simulink model "pcssp_controller_and_ps_psc"  (R2025b)
settings: Solver=VariableStepAuto  StartTime=t_start  StopTime=t_max  RelTol=1e-3
values from neighbouring files (symbols this model uses):
  AllocatorMode = 1    [muscle_controller_NICE_IMAS_iter_init.m]    (also in muscle_controller_NICE_IMAS_iter_init_psc.m)
  enable_KCURR = double(instance.get_setting('KCURR', pyargs('default', 1)))    [muscle_controller_NICE_IMAS_iter_init.m]    (also in muscle_controller_NICE_IMAS_iter_init_psc.m)
  enable_RZIp = double(instance.get_setting('RZIp', pyargs('default', 0)))    [muscle_controller_NICE_IMAS_iter_init.m]    (also in muscle_controller_NICE_IMAS_iter_init_psc.m)
  enable_VS = double(instance.get_setting('VS', pyargs('default', 1)))    [muscle_controller_NICE_IMAS_iter_init.m]    (also in muscle_controller_NICE_IMAS_iter_init_psc.m)
  in_out_dt = double(instance.get_setting('in_out_msg_dt', pyargs('default', 0.001)))    [muscle_controller_NICE_IMAS_iter_init.m]    (also in muscle_controller_NICE_IMAS_iter_init_psc.m)
  IpControlMode = 0    [muscle_controller_NICE_IMAS_iter_init.m]    (also in muscle_controller_NICE_IMAS_iter_init_psc.m)
  IpControlMode_KCURR = double(instance.get_setting('control_Ip', pyargs('default', 1)))    [muscle_controller_NICE_IMAS_iter_init.m]    (also in muscle_controller_NICE_IMAS_iter_init_psc.m)
  IpControlMode_RZIp = 0    [muscle_controller_NICE_IMAS_iter_init.m]    (also in muscle_controller_NICE_IMAS_iter_init_psc.m)
  SchedulingVar_GapContr = 0    [muscle_controller_NICE_IMAS_iter_init.m]    (also in muscle_controller_NICE_IMAS_iter_init_psc.m)
  schedulingVar_KCURR = 0    [muscle_controller_NICE_IMAS_iter_init.m]    (also in muscle_controller_NICE_IMAS_iter_init_psc.m)
  SCIpScaling = 0    [muscle_controller_NICE_IMAS_iter_init.m]    (also in muscle_controller_NICE_IMAS_iter_init_psc.m)
  ShapeIpControlMode = double(instance.get_setting('Shape_control', pyargs('default', 0)))    [muscle_controller_NICE_IMAS_iter_init.m]    (also in muscle_controller_NICE_IMAS_iter_init_psc.m)
  usePSModel = double(instance.get_setting('PSModel', pyargs('default', 1)))    [muscle_controller_NICE_IMAS_iter_init.m]    (also in muscle_controller_NICE_IMAS_iter_init_psc.m)
  VSControlMode = double(instance.get_setting('VS_control_mode', pyargs('default', 3)))    [muscle_controller_NICE_IMAS_iter_init.m]    (also in muscle_controller_NICE_IMAS_iter_init_psc.m)
  VSIpScaling = 1    [muscle_controller_NICE_IMAS_iter_init.m]    (also in muscle_controller_NICE_IMAS_iter_init_psc.m)
Description:
  | The KCURR_PFPO1 module implements a CS/PF current controller, including control of IpThis version performs internal gain scheduling based on an externally fed scheduling variable. Note: the coils are sorted as CS3U CS2U CS1 CS2L CS3L P1 P2 P3 P4 P5 P6
settings Model: DataDictionary=pcssp_controller_and_ps_psc.sldd  VariantFading=off  Creator=ravenst1  LastModifiedBy=schneim
settings SolverCC: AutoInsertRateTranBlk=on
settings DebuggingCC: UnderspecifiedInitializationDetection=Classic  MergeDetectMultiDrivingBlocksExec=none
settings ModelReferenceCC: PropagateSignalLabelsOutOfModel=off

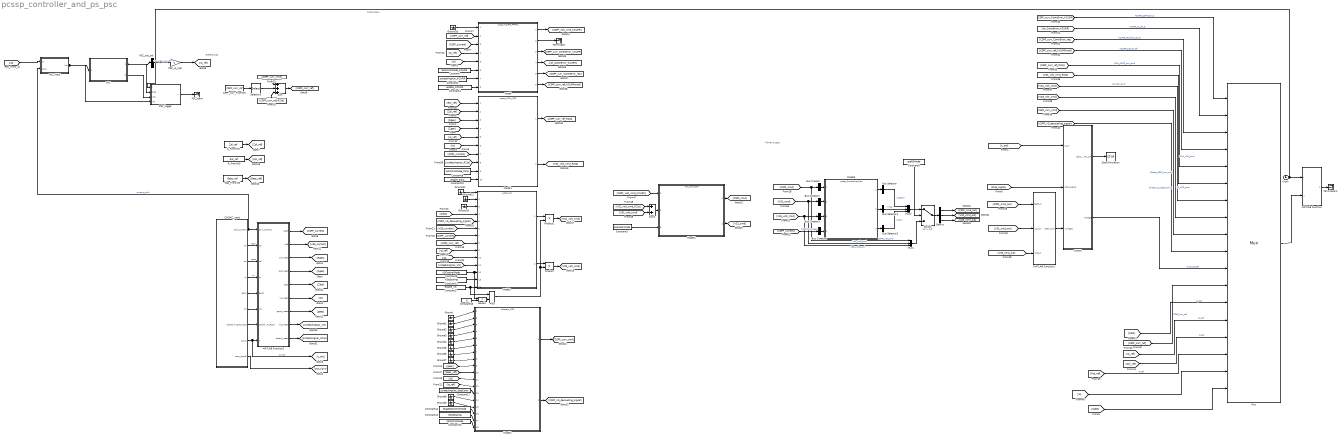
== system pcssp_controller_and_ps_psc ==
  note: Power supply
  note: Controllers
  note: References
  AND : Logic  IconShape=distinctive  AllPortsSameDT=off  OutDataTypeStr=boolean
  Bus Creator : BusCreator  Inputs=1  OutDataTypeStr=Bus:pcssp_PS_CSPF_volt_cmd
  Bus Creator2 : BusCreator  Inputs=1  OutDataTypeStr=Bus: pcssp_PS_VS1_volt_cmd
  Bus Creator3 : BusCreator  Inputs=1  OutDataTypeStr=Bus: pcssp_PS_VS3_volt_cmd
  Bus Creator4 : BusCreator  Inputs=1  OutDataTypeStr=Bus: pcssp_PS_CSPF_curr_meas
  Bus Selector : BusSelector  OutputSignals=VCSPF
  Bus Selector1 : BusSelector  OutputSignals=VS1
  Bus Selector2 : BusSelector  OutputSignals=VS3
  CODAC_input : MATLAB Function  TreatAsAtomicUnit=on  SystemSampleTime=in_out_dt
  CSPF_curr_FromWS : FromWorkspace  VariableName=CSPF_curr_ref
  Clock : Clock
  Constant : Constant  Value=IpControlMode_KCURR  OutDataTypeStr=boolean
  Constant1 : Constant  Value=schedulingVar_KCURR
  Constant10 : Constant  Value=enable_RZIp  OutDataTypeStr=boolean
  Constant11 : Constant  Value=VSIpScaling
  Constant12 : Constant  Value=SCIpScaling
  Constant13 : Constant  Value=IpControlMode
  Constant14 : Constant  Value=ShapeIpControlMode
  Constant15 : Constant  Value=0
  Constant17 : Constant  Value=SchedulingVar_GapContr
  Constant2 : Constant  Value=enable_VS  OutDataTypeStr=boolean
  Constant3 : Constant  Value=AllocatorMode
  Constant4 : Constant  Value=enable_KCURR
  Constant5 : Constant  Value=usePSModel
  Constant6 : Constant  Value=VSControlMode
  Constant8 : Constant  Value=IpControlMode_RZIp  OutDataTypeStr=boolean
  Demux : Demux  Outputs=[11 1 1]
  Equal4 : RelationalOperator  Operator=>  OutDataTypeStr=boolean  RndMeth=Simplest  InputSameDT=off
  Gap_FromWS : FromWorkspace  VariableName=Gaps_ref
  Ground{,1..13} (14 alike) : Ground
  MATLAB Function : MATLAB Function  TreatAsAtomicUnit=on  SystemSampleTime=in_out_dt
  MATLAB Function1 : MATLAB Function  TreatAsAtomicUnit=on  SystemSampleTime=in_out_dt
  MATLAB Function2 : MATLAB Function  TreatAsAtomicUnit=on  SystemSampleTime=in_out_dt
  Model : ModelReference  ModelNameDialog=pcssp_KCURR_PFPO1.slx  SimulationMode=Normal  ModelReferenceVersion=6.1
  Model1 : ModelReference  ModelNameDialog=pcssp_RZIp_CCS.slx  SimulationMode=Normal  ModelReferenceVersion=10.5
  Model2 : ModelReference  ModelNameDialog=shapeIp_CCS.slx  SimulationMode=Normal  ModelReferenceVersion=1.1
  Model3 : ModelReference  ModelNameDialog=pcssp_VS.slx  SimulationMode=Normal  ModelReferenceVersion=7.2
  Model4 : ModelReference  ModelNameDialog=VS1_allocator.slx  SimulationMode=Normal  ModelReferenceVersion=1.4
  Model5 : ModelReference  ModelNameDialog=pcssp_PowerSupplies.slx  ParameterArgumentNames=PS_tp  UsingDefaultArgumentValue=0  SimulationMode=Normal  ModelReferenceVersion=1.39
  Mux : Mux  Inputs=18
      settings: DisplayOption=signals
  Mux1 : Mux  Inputs=3
  Mux2 : Mux  Inputs=3
  Output : MATLAB Function  TreatAsAtomicUnit=on  SystemSampleTime=in_out_dt
  PSC : Subsystem  ReferencedSubsystem=PSC  ConfFolderPath=/Users/igo/Data_Igor_Local/GitFolder/pcs  PSCInterConfFileName=[]  GlobMonFileName=[]  DecisionFileName=[]  RefGenFileName=[]  useInBus=Bus signal  useInPorts=Ports  useOutBus=Bus signal  useOutPorts=Ports  SaveStatus=off
  PSC_Ip_sign : Gain  Gain=-1
  PSC_input : MATLAB Function  TreatAsAtomicUnit=on
  PSC_logger : MATLAB Function  TreatAsAtomicUnit=on
  PSC_out_sel : BusSelector  OutputSignals=psc_ref__Ipl_ref
  PSC_term : Terminator
  Product : Product
  Product1 : Product
  R_FromWS : FromWorkspace  VariableName=Rpl_ref
  Selector3 : Selector  IndexMode=Zero-based  InputPortWidth=14  IndexOptions=Index vector (dialog)  Indices=[0 1 2 4 5 6 7 8 9 10 11]  OutputSizes=1
  Stop Simulation : Stop
  Sum : Sum  Inputs=+++
  Sum1 : Sum
  Switch : Switch  Criteria=u2 > Threshold  Threshold=0.5  SaturateOnIntegerOverflow=off  InputSameDT=off
  Terminator : Terminator
  Terminator2 : Terminator
  Z_FromWS : FromWorkspace  VariableName=Zpl_ref
  wires:
  CODAC_input/1(coils_current) -> MATLAB Function2/1(coil_currents), PSC_input/2(coils)  "current_coils"
  Model/1 -> [CSPF_volt_cmd_KCURR]
  Constant1/1 -> Model/7
  Constant/1 -> Model/6
  Constant8/1 -> Model1/9
  [schedulingVar_RZIp] -> Model1/8
  CSPF_curr_FromWS/1 -> Selector3/1
  Model/2 -> Terminator/1
  Model1/1 -> [CSPF_curr_ref_RZIp]
  Output/1(stop_signal_out) -> Stop Simulation/1
  [Rpl_ref] -> Model1/1
  [Zgeo] -> Model1/4
  [Rgeo] -> Model1/3
  [Ip] -> Model/5
  [t_out] -> Output/1(t_cur)
  [stop_signal] -> Output/2(stop_signal)
  CODAC_input/9(stop_signal) -> [stop_signal]
  [CSPF_current] -> Model/3
  [CSPF_current] -> Model1/7
  Z_FromWS/1 -> [Zpl_ref]
  [Zpl_ref] -> Model1/2
  Ground11/1 -> Model3/1
  [Ip_ref] -> Model/4
  [schedulingVar_VS] -> Model3/11
  Constant6/1 -> Equal4/1, Model3/12
  [CSPF_curr_ref] -> Model/2
  [Zdot] -> Model3/4
  Constant11/1 -> Model3/13
  Gap_FromWS/1 -> [Gaps_ref]
  Model1/2 -> [VS1_volt_cmd_RZIp]
  Equal4/1 -> AND/2
  Constant15/1 -> Equal4/2
  Model3/2 -> Product/1
  Product/1 -> [VS3_volt_cmd]
  AND/1 -> Product1/2, Product/2
  Product1/1 -> [VS1_volt_cmd]
  Model3/1 -> Product1/1
  R_FromWS/1 -> [Rpl_ref]
  [CSPF_current] -> Model3/7
  [VS3_current] -> Model3/6
  [CSPF_curr_ref] -> Model3/8
  Model2/1 -> [CSPF_curr_cmd]
  [CSPF_curr_cmd] -> Sum/1
  [CSPF_curr_ref_RZIp] -> Sum/3
  Sum/1 -> [CSPF_curr_ref]
  [Ip_ref] -> Model2/12
  [gaps] -> Model2/9
  Ground5/1 -> Model2/6
  Ground9/1 -> Model2/15
  Ground8/1 -> Model2/14
  [Ip] -> Model2/11
  [Gaps_ref] -> Model2/10
  Ground1/1 -> Model2/2
  Ground3/1 -> Model2/4
  Constant12/1 -> Model2/17
  Constant17/1 -> Model2/13
  Ground/1 -> Model2/1
  Model2/2 -> [CSPF_VS_decoupling_signal]
  Ground7/1 -> Model2/8
  Ground2/1 -> Model2/3
  Ground6/1 -> Model2/7
  Ground4/1 -> Model2/5
  Constant14/1 -> Model2/16
  [CSPF_VS_decoupling_signal] -> Model3/5
  Model/6 -> [CSPF_curr_ref_KCURRmod]
  Model/5 -> [CSPF_curr_ContrError_res]
  Model/4 -> [Ipl_ContrError_KCURR]
  Model/3 -> [CSPF_curr_ContrError_KCURR]
  Constant10/1 -> Model1/10
  Constant4/1 -> Model/8
  Constant2/1 -> AND/1, Model3/14
  Constant13/1 -> Model2/18
  [Ip_ref] -> Model3/9
  [Ip] -> Model3/10
  [Ip_ref] -> Model1/5
  [Ip] -> Model1/6
  Ground10/1 -> Model/1
  Ground12/1 -> Model3/2
  Ground13/1 -> Model3/3
  Selector3/1 -> Sum/2
  MATLAB Function/1(y) -> Terminator2/1
  Clock/1 -> MATLAB Function/1(t), PSC_logger/1(t)
  Output/2(voltage) -> Mux/11  "Output_total"
  [CSPF_curr_ContrError_KCURR] -> Mux/1  "KCURR_CSPF_ctrl_e"
  [Ipl_ContrError_KCURR] -> Mux/2  "KCURR_Ip_ctrl_e"
  [CSPF_curr_ContrError_res] -> Mux/3  "KCURR_residual_ctrl_e"
  [CSPF_curr_ref_KCURRmod] -> Mux/4  "KCURR_actual_ref"
  [CSPF_curr_ref_RZIp] -> Mux/5  "RZIp_CSPF_curr_cmd"
  [VS1_volt_cmd_RZIp] -> Mux/6  "RZIp_VS1_cmd"
  [VS1_volt_cmd] -> Mux/7  "VS_VS1_cmd"
  [VS3_volt_cmd] -> Mux/8  "VS_VS3_cmd"
  [CSPF_curr_cmd] -> Mux/9  "Shape_CSPF_curr_cmd"
  [CSPF_VS_decoupling_signal] -> Mux/10  "Shape_VS_decoupling"
  Mux/1 -> MATLAB Function/2(u)
  [CSPF_curr_ref] -> Mux/12  "CSPF_curr_ref"
  [Ip_ref] -> Mux/14  "Ip_ref"
  [Zpl_ref] -> Mux/15  "Z_ref"
  [Rpl_ref] -> Mux/16  "R_ref"
  [Zdot] -> Mux/13  "Z_dot"
  [Ip] -> Mux/17
  [CSPF_volt_cmd_KCURR] -> Model4/1
  [VS1_volt_cmd_RZIp] -> Sum1/1
  [VS1_volt_cmd] -> Sum1/2
  Sum1/1 -> Model4/2
  Model4/2 -> [VS1_cmd]
  Model4/1 -> [CSPF_cmd]
  Constant3/1 -> Model4/3
  CODAC_input/2(rpl) -> MATLAB Function2/2(rpl)  "rgeo"
  CODAC_input/3(zpl) -> MATLAB Function2/3(zpl)  "zgeo"
  CODAC_input/4(ip) -> MATLAB Function2/4(ip)  "ip"
  CODAC_input/5(gaps) -> MATLAB Function2/5(gaps)
  CODAC_input/6(li3) -> MATLAB Function2/6(li3)
  CODAC_input/7(schedulingVar_RZIp) -> MATLAB Function2/7(schedulingVar_RZIp)
  CODAC_input/8(t_out) -> MATLAB Function2/8(t), [t_out]  "t_msg"
  MATLAB Function2/1(Icspf) -> [CSPF_current]
  MATLAB Function2/2(Ivs3) -> [VS3_current]
  MATLAB Function2/3(rpl_meas) -> [Rgeo]
  MATLAB Function2/4(zpl_meas) -> [Zgeo]
  MATLAB Function2/5(zdot) -> [Zdot]
  MATLAB Function2/6(ip_meas) -> [Ip]
  MATLAB Function2/7(gaps_meas) -> [gaps]
  MATLAB Function2/9(sched_meas) -> [schedulingVar_RZIp]
  MATLAB Function2/8(li3_meas) -> [schedulingVar_VS]
  MATLAB Function1/1(total_cmd) -> Output/3("voltage ")
  [CSPF_cmd_out] -> MATLAB Function1/1(cspfout)
  [VS1_cmd_out] -> MATLAB Function1/2(vs1out)
  [VS3_cmd_out] -> MATLAB Function1/3(vs3out)
  [CSPF_cmd] -> Mux1/1, Bus Creator/1  "CSPF_volt_cmd"
  Bus Creator/1 -> Model5/1
  Bus Creator2/1 -> Model5/2
  [VS1_cmd] -> Mux1/2, Bus Creator2/1  "VS1_volt_cmd"
  [VS3_volt_cmd] -> Mux1/3, Bus Creator3/1  "VS3_volt_cmd"
  Bus Creator3/1 -> Model5/3
  [CSPF_current] -> Bus Creator4/1  "CSPF_curr_meas"
  Bus Creator4/1 -> Model5/4
  Model5/1 -> Bus Selector/1
  Bus Selector/1 -> Mux2/1  "<VCSPF>"
  Bus Selector1/1 -> Mux2/2  "<VS1>"
  Model5/2 -> Bus Selector1/1
  Model5/3 -> Bus Selector2/1
  Bus Selector2/1 -> Mux2/3  "<VS3>"
  Mux2/1 -> Switch/1
  Mux1/1 -> Switch/3
  Constant5/1 -> Switch/2
  Switch/1 -> Demux/1
  Demux/1 -> [CSPF_cmd_out]
  Demux/2 -> [VS1_cmd_out]
  Demux/3 -> [VS3_cmd_out]
  [Zgeo] -> Mux/18
  [Ip] -> PSC_input/1(ip)
  PSC_input/1(inb) -> PSC/1, PSC_logger/4(inb)
  PSC/1 -> PSC_out_sel/1, PSC_logger/2(outb)
  PSC_out_sel/1 -> PSC_Ip_sign/1  "<psc_ref__Ipl_ref>"
  PSC_Ip_sign/1 -> [Ip_ref]
  PSC/2 -> PSC_logger/3(intb)
  PSC_logger/1(y) -> PSC_term/1

== matlab function pcssp_controller_and_ps_psc/MATLAB Function ==
  data: t input; u input; y output
function y = csv_logger(t,u)
coder.extrinsic('log_row');
log_row(t, u);
y = 0;
end

== matlab function pcssp_controller_and_ps_psc/PSC_input ==
  data: ip input; inb output Bus: PSC_In_Bus; coils input
function inb = psc_input(ip, coils)
% PSC-4: PSC_In_Bus from the measurements of the glue (PCS frame, SI units).
coder.extrinsic('psc_zgeo_get');
z = 0;
z = psc_zgeo_get();
inb.ip_ip__meas.value = -ip;
inb.ip_ip__meas.quality = PcsQuality_t.kGood;
inb.ip_ip__meas.activity = PcsActivity_t.kRunning;
inb.plasma_state__exist_diag.value = 1;
inb.plasma_state__exist_diag.quality = PcsQuality_t.kGood;
inb.plasma_state__exist_diag.activity = PcsActivity_t.kRunning;
inb.z_meas.value = z;
inb.z_meas.quality = PcsQuality_t.kGood;
inb.z_meas.activity = PcsActivity_t.kRunning;
inb.cs_margin.value = min(45e3 - abs(coils(1:6)));
inb.cs_margin.quality = PcsQuality_t.kGood;
inb.cs_margin.activity = PcsActivity_t.kRunning;
end

== matlab function pcssp_controller_and_ps_psc/Output ==
  data: t_cur input; stop_signal input; voltage input; stop_signal_out output; voltage output
function [stop_signal_out, voltage] = CODAC_output(t_cur, stop_signal,voltage)



% constrain python function to run extrinsically in Matlab (no codegen)
coder.extrinsic('muscle_control2nice');

muscle_control2nice(t_cur,voltage);

stop_signal_out = stop_signal;

== matlab function pcssp_controller_and_ps_psc/PSC_logger ==
  data: t input; y output; outb input Bus: PSC_Out_Bus; intb input Bus: PSC_Int_Bus; inb input Bus: PSC_In_Bus
function y = psc_logger(t, outb, intb, inb)
% PSC-4: one row per tick into RUN_DIR/psc_log.csv (psc_log_row.m, header written by the glue).
coder.extrinsic('psc_log_row');
u = [outb.psc_ref__Ipl_ref; double(intb.psc_ref__current_segment); double(intb.psc_ref_lastModSegment); ...
     double(intb.psc_OldModSegment); intb.psc_segmentTime; intb.psc_simTime; intb.psc_lastTimeDiff; ...
     double(intb.glb_ps__run_plasma); double(intb.glb__PulseDone); double(intb.glb_ps__ip_too_high); ...
     double(intb.glb_ps__end_of_flux); double(intb.glb_ps__z_excursion); ...
     inb.ip_ip__meas.value; inb.z_meas.value; inb.cs_margin.value];
psc_log_row(t, u);
y = 0;
end

== matlab function pcssp_controller_and_ps_psc/CODAC_input ==
  data: coils_current output; rpl output; zpl output; ip output; gaps output; li3 output; schedulingVar_RZIp output; t_out output; stop_signal output
function [coils_current,rpl,zpl,ip,gaps,li3,schedulingVar_RZIp,t_out,stop_signal] = CODAC_input
% Receives the plant measurements from MUSCLE3 (muscle_nice2control, run in MATLAB).

% outputs of an extrinsic call: size and type must be declared beforehand
N_GAPS = 62;
coils_current = zeros(14,1);
rpl = 0;
zpl = 0;
ip = 0;
gaps = zeros(N_GAPS,1);
li3 = 0;
schedulingVar_RZIp = zeros(3,1);
t_out = 0;
stop_signal = 0;

% runs in MATLAB, not compiled (it calls MUSCLE3 through Python)
coder.extrinsic('muscle_nice2control');

[coils_current,rpl,zpl,ip,gaps,li3,schedulingVar_RZIp,t_out,stop_signal] = muscle_nice2control();
end

== matlab function pcssp_controller_and_ps_psc/MATLAB Function1 ==
  data: cspfout input; total_cmd output; vs1out input; vs3out input
function total_cmd = output_block(cspfout, vs1out, vs3out)
    coder.extrinsic('controller_output_preprocess');
    total_cmd = zeros(14,1);
    total_cmd = controller_output_preprocess(cspfout, vs1out, vs3out);
end

== matlab function pcssp_controller_and_ps_psc/MATLAB Function2 ==
  data: coil_currents input; Icspf output; rpl input; zpl input; ip input; gaps input; li3 input; schedulingVar_RZIp input; t input; Ivs3 output; rpl_meas output; zpl_meas output; zdot output; ip_meas output; gaps_meas output; li3_meas output; sched_meas output
function [Icspf,Ivs3,rpl_meas,zpl_meas,zdot,ip_meas,gaps_meas,li3_meas,sched_meas] = preprocess_block(coil_currents,rpl,zpl,ip,gaps,li3,schedulingVar_RZIp,t)

coder.extrinsic('controller_input_preprocess');

% outputs of an extrinsic call: size and type must be declared beforehand
Icspf = zeros(11,1);
Ivs3  = 0;
rpl_meas = 0;  zpl_meas = 0;  zdot = 0;  ip_meas = 0;  li3_meas = 0;
gaps_meas  = zeros(size(gaps));
sched_meas = zeros(size(schedulingVar_RZIp));

[Icspf,Ivs3,rpl_meas,zpl_meas,zdot,ip_meas,gaps_meas,li3_meas,sched_meas] = ...
    controller_input_preprocess(coil_currents,rpl,zpl,ip,gaps,li3,schedulingVar_RZIp,t);
end
